simulink model "Invert_Pendulum"  (R2025a)
settings: Solver=VariableStepAuto  StartTime=0.0  StopTime=5  RelTol=1e-3
values from neighbouring files (symbols this model uses):
  g = 9.81    [transfer_fcn.m]
  J = m * L^2 / 3    (= 14.45)    [transfer_fcn.m]
  L = 1.7/2    (= 0.85)    [transfer_fcn.m]
  m = 60    [transfer_fcn.m]
  M = 47.7    [transfer_fcn.m]
libraries: slpidlib x1
settings Model: Creator=yiqun  LastModifiedBy=yiqun

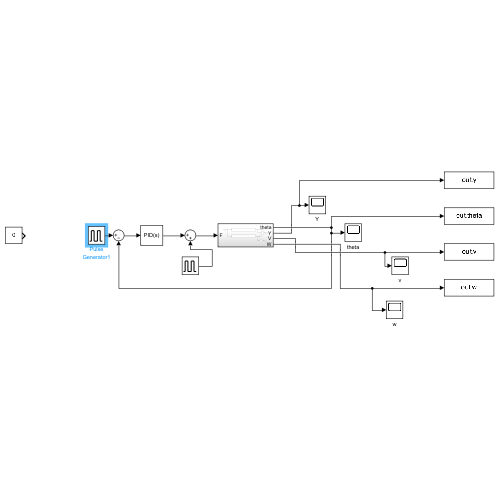
[thumbnail: Simulink's stored preview of the top-level diagram]
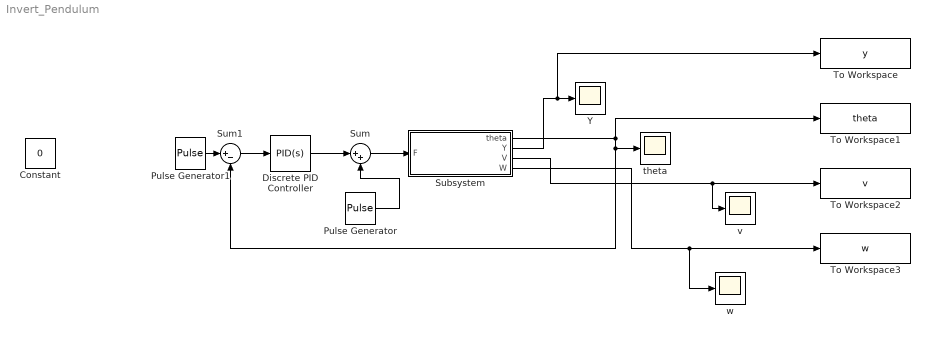
== system Invert_Pendulum ==
  Constant : Constant  Value=0
  Discrete PID Controller : slpidlib/PID Controller  Controller=PID  Form=Parallel  TimeDomain=Continuous-time  UseExternalTs=off  SampleTime=-1  IntegratorMethod=Forward Euler  FilterMethod=Forward Euler  ControllerParametersSource=internal  P=-20000  I=-30000  UseKiTs=off  D=-6000  UseExternalDerivativeSource=off  N=100  UseFilter=on  TunerSelectOption=Transfer Function Based (PID Tuner App)  InitialConditionSource=internal  InitialConditionForIntegrator=0  InitialConditionForFilter=0  DifferentiatorICPrevScaledInput=0  ExternalReset=none  TrackingMode=off  Kt=1  LimitOutput=off  SatLimitsSource=internal  UpperSaturationLimit=inf  LowerSaturationLimit=-inf  LinearizeAsGain=off  AntiWindupMode=none  Kb=1  LimitIntegrator=off  UpperIntegratorSaturationLimit=inf  LowerIntegratorSaturationLimit=-inf  POutMin=[]  POutMax=[]  IOutMin=[]  IOutMax=[]  DOutMin=[]  DOutMax=[]  NOutMin=[]  NOutMax=[]  SumOutMin=[]  SumOutMax=[]  SaturationOutMin=[]  SaturationOutMax=[]  PParamMin=[]  PParamMax=[]  IParamMin=[]  IParamMax=[]  DParamMin=[]  DParamMax=[]  NParamMin=[]  NParamMax=[]  KbParamMin=[]  KbParamMax=[]  KtParamMin=[]  KtParamMax=[]  KbOutMin=[]  KbOutMax=[]  KtOutMin=[]  KtOutMax=[]  IntegratorOutMin=[]  IntegratorOutMax=[]  FilterOutMin=[]  FilterOutMax=[]  SumI1OutMin=[]  SumI1OutMax=[]  SumI2OutMin=[]  SumI2OutMax=[]  SumI3OutMin=[]  SumI3OutMax=[]  SumI4OutMin=[]  SumI4OutMax=[]  SumDOutMin=[]  SumDOutMax=[]  DifferentiatorOutMin=[]  DifferentiatorOutMax=[]  FilterDiffOutCoefMin=[]  FilterDiffOutCoefMax=[]  ReciprocalOutMin=[]  ReciprocalOutMax=[]  SumDenOutMin=[]  SumDenOutMax=[]  SumNumOutMin=[]  SumNumOutMax=[]  DivideOutMin=[]  DivideOutMax=[]  UdiffTsProdOutMin=[]  UdiffTsProdOutMax=[]  NTsProdOutMin=[]  NTsProdOutMax=[]  UintegralTsProdOutMin=[]  UintegralTsProdOutMax=[]  UngainTsProdOutMin=[]  UngainTsProdOutMax=[]  ClampingZeroOutDataTypeStr=Inherit: Inherit via back propagation  ClampingZeroOutMin=[]  ClampingZeroOutMax=[]  FilterDenConstantOutDataTypeStr=Inherit: Inherit via back propagation  FilterDenConstantOutMin=[]  FilterDenConstantOutMax=[]  PCopyOutDataTypeStr=Inherit: Inherit via back propagation  PCopyOutMin=[]  PCopyOutMax=[]  NCopyOutDataTypeStr=Inherit: Inherit via back propagation  NCopyOutMin=[]  NCopyOutMax=[]  IntegratorContinuousStateAttributes=''  IntegratorStateMustResolveToSignalObject=off  IntegratorRTWStateStorageClass=Auto  FilterContinuousStateAttributes=''  FilterStateMustResolveToSignalObject=off  FilterRTWStateStorageClass=Auto  ParallelPVariant=InternalParameters  IdealPVariant=Disabled  IVariant=InternalParameters  DVariant=InternalParameters  IntegratorVariant=Continuous  SatVariant=Disabled  AWVariant=Passthrough  PCopyVariant=Disabled  TRVariant=Disabled  FdbkBlocksVariant=Forward  IdealPFdbkVariant=Disabled  SatFdbkVariant=Disabled  DerivativeFilterVariant=ContFilter  NVariant=InternalParameters  NCopyVariant=Disabled  FilterICVariant=InternalICsFilter  IntegratorICVariant=InternalICs  ExternalResetVariant=Disabled  TRSumVariant=Passthrough  SumFdbkVariant=Disabled  SumVariant=Sum_PID  TsampFilterVariant=InternalTs  TsampNgainVariant=Passthrough  TsampIntegralVariant=Disabled_SignalSpec  ExternalSaturationOutDataTypeStr=Inherit: Same as second input  DerivativeSourceVariant=ErrorSignal  PreIntVariant=InternalPreInt
      settings: LibrarySourceBlock=simulink/Discrete/Discrete PID Controller
  Pulse Generator : DiscretePulseGenerator  PulseType=Time based  Amplitude=5e4  Period=1
  Pulse Generator1 : DiscretePulseGenerator  PulseType=Time based  Amplitude=-20/180 *3.14  Period=1  PhaseDelay=0.2
  Subsystem : Subsystem
  Sum : Sum  Inputs=|++
  Sum1 : Sum  Inputs=|+-
  To Workspace : ToWorkspace  VariableName=y  SampleTime=-1
  To Workspace1 : ToWorkspace  VariableName=theta  SampleTime=-1
  To Workspace2 : ToWorkspace  VariableName=v  SampleTime=-1
  To Workspace3 : ToWorkspace  VariableName=w  SampleTime=-1
  Y : Scope
      settings: ActiveDisplayYMinimum=-62.351020636190086  ActiveDisplayYMaximum=20.489945610913608
  theta : Scope
      settings: ActiveDisplayYMinimum=-0.64061519382432541  ActiveDisplayYMaximum=0.24747823729346929
  v : Scope
      settings: ActiveDisplayYMinimum=-7.3927981733013066  ActiveDisplayYMaximum=9.7975023352161656  DataLoggingVariableName=ScopeData2
  w : Scope
      settings: ActiveDisplayYMinimum=-10.582579601999077  ActiveDisplayYMaximum=12.593549188975659  DataLoggingVariableName=ScopeData3
  wires:
  Pulse Generator/1 -> Sum/2
  Discrete PID Controller/1 -> Sum/1
  Sum1/1 -> Discrete PID Controller/1
  Sum/1 -> Subsystem/1(F)
  Subsystem/1(theta) -> Sum1/2, theta/1, To Workspace1/1
  Subsystem/2(Y) -> To Workspace/1, Y/1
  Subsystem/3(V) -> v/1, To Workspace2/1
  Subsystem/4(W) -> w/1, To Workspace3/1
  Pulse Generator1/1 -> Sum1/1

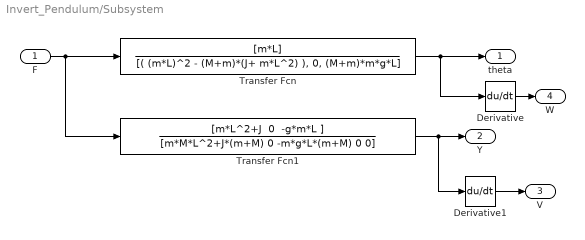
== system Invert_Pendulum/Subsystem ==
  F : Inport
  Derivative : Derivative
  Derivative1 : Derivative
  Transfer Fcn : TransferFcn  Numerator=[m*L]  Denominator=[( (m*L)^2 - (M+m)*(J+ m*L^2) ), 0, (M+m)*m*g*L]
  Transfer Fcn1 : TransferFcn  Numerator="[m*L^2+J  0  -g*m*L ]"  Denominator=[m*M*L^2+J*(m+M) 0 -m*g*L*(m+M) 0 0]
  theta : Outport
  Y : Outport  Port=2
  V : Outport  Port=3
  W : Outport  Port=4
  wires:
  Transfer Fcn/1 -> Derivative/1, theta/1
  F/1 -> Transfer Fcn1/1, Transfer Fcn/1
  Transfer Fcn1/1 -> Derivative1/1, Y/1
  Derivative/1 -> W/1
  Derivative1/1 -> V/1
